simulink model "gtm_design"  (R2021b)
settings: Solver=VariableStepAuto  StartTime=0.0  StopTime=10.0  MinStep=0.00999  RelTol=1e-3
StopFcn:
  | MWSout=grabmws(bdroot);
  | MWSout.lastrun=datestr(now);
values from neighbouring files (symbols this model uses):
  knots2fps = 1.68781    [setup.m]
  s = tf('s')    [setup.m]
undefined symbols (not defined in the file or in its folder): Aero, aftfuel, aftfuel_pos, AILL, AILLC, AILR, AILRC, alpha_deg, alt0, altitude_ft, Ax_g, Ay_g, Az_g, b, beta_deg, bias, BRAKEC, Cbar, cg_pos0, cg_shift_gear, ControlMode, DamageCase, DamageModels, DamageOnsetTime, deltc, Earth, ELLIB, ELLIBC, ELLOB, ELLOBC, ELRIB, ELRIBC, ELROB, ELROBC, engl_ang, engl_pos, engr_ang, engr_pos, etas0, etas1, etasc_feedthrough, FLAPLC, FLAPLIB, FLAPLOB, FLAPRC, FLAPRIB, FLAPROB, FlightMode, FuelUsed_Init, fwdfuel, fwdfuel_pos, GEAR, GEARC, Inertia0, Inertia_shift_gear, Ixx_model, Iyy_model, Izz_model, KTAS, LandingGear ... (+66)
libraries: simulink_extras x98, LPVBlockLibrary x54, simulink_need_slupdate x30, aerolibconvert2 x27, simulink x7, aerolibtransform2 x6, uavalgslib x4, UserContent_lib x2, robotcorelib x1, uavutilslib x1
(part 8 of 9)

== system gtm_design/GTM_T2/Aero/Control Surfaces/Spoilers/InboardSpoilers ==
  alpha : Inport
  beta : Inport  Port=2
  SPLLIB : Inport  Port=3
  SPLRIB : Inport  Port=4
  Constant1 : Constant  Value=[0:5]  OutDataTypeStr=uint32
  Constant3 : Constant  Value=[0:5]  OutDataTypeStr=uint32
  Gain2 : Gain  Gain=-1
  Interpolation Using Prelookup : Interpolation_n-D  NumberOfTableDimensions=4  Table=Aero.dC6_spo.data  NumSelectionDims=1
      settings: InputPortMap=u0,u1,u2,u3,u4,u5,u6
  Interpolation Using Prelookup1 : Interpolation_n-D  NumberOfTableDimensions=4  Table=Aero.dC6_spo.data  NumSelectionDims=1
      settings: InputPortMap=u0,u1,u2,u3,u4,u5,u6
  Negate Lateral : Gain  Gain=[1 -1 1 -1 1 -1]
  Prelookup1 : PreLookup  BreakpointsData=Aero.dC6_spo.alpha  IndexSearchMethod=Linear search  BeginIndexSearchUsingPreviousIndexResult=on  ExtrapMethod=Linear
  Prelookup2 : PreLookup  BreakpointsData=Aero.dC6_spo.beta  IndexSearchMethod=Linear search  BeginIndexSearchUsingPreviousIndexResult=on  ExtrapMethod=Linear
  Prelookup3 : PreLookup  BreakpointsData=Aero.dC6_spo.spo  IndexSearchMethod=Linear search  BeginIndexSearchUsingPreviousIndexResult=on  ExtrapMethod=Linear
  Prelookup4 : PreLookup  BreakpointsData=Aero.dC6_spo.beta  IndexSearchMethod=Linear search  BeginIndexSearchUsingPreviousIndexResult=on  ExtrapMethod=Linear
  Prelookup5 : PreLookup  BreakpointsData=Aero.dC6_spo.spo  IndexSearchMethod=Linear search  BeginIndexSearchUsingPreviousIndexResult=on  ExtrapMethod=Linear
  Left : Outport
  Right : Outport  Port=2
  wires:
  Gain2/1 -> Prelookup2/1
  Negate Lateral/1 -> Left/1
  Interpolation Using Prelookup1/1 -> Right/1
  SPLRIB/1 -> Prelookup5/1
  beta/1 -> Gain2/1, Prelookup4/1
  alpha/1 -> Prelookup1/1
  SPLLIB/1 -> Prelookup3/1
  Prelookup1/1 -> Interpolation Using Prelookup/1, Interpolation Using Prelookup1/1
  Prelookup1/2 -> Interpolation Using Prelookup/2, Interpolation Using Prelookup1/2
  Prelookup2/1 -> Interpolation Using Prelookup/3
  Prelookup2/2 -> Interpolation Using Prelookup/4
  Prelookup3/1 -> Interpolation Using Prelookup/5
  Prelookup3/2 -> Interpolation Using Prelookup/6
  Constant3/1 -> Interpolation Using Prelookup/7
  Prelookup4/1 -> Interpolation Using Prelookup1/3
  Prelookup4/2 -> Interpolation Using Prelookup1/4
  Prelookup5/1 -> Interpolation Using Prelookup1/5
  Prelookup5/2 -> Interpolation Using Prelookup1/6
  Constant1/1 -> Interpolation Using Prelookup1/7
  Interpolation Using Prelookup/1 -> Negate Lateral/1

== system gtm_design/GTM_T2/Aero/Control Surfaces/Spoilers/OutboardSpoilers ==
  alpha : Inport
  beta : Inport  Port=2
  SPLLIB : Inport  Port=3
  SPLRIB : Inport  Port=4
  Constant1 : Constant  Value=[0:5]  OutDataTypeStr=uint32
  Constant3 : Constant  Value=[0:5]  OutDataTypeStr=uint32
  Gain2 : Gain  Gain=-1
  Interpolation Using Prelookup : Interpolation_n-D  NumberOfTableDimensions=4  Table=Aero.dC6_spo.data  NumSelectionDims=1
      settings: InputPortMap=u0,u1,u2,u3,u4,u5,u6
  Interpolation Using Prelookup1 : Interpolation_n-D  NumberOfTableDimensions=4  Table=Aero.dC6_spo.data  NumSelectionDims=1
      settings: InputPortMap=u0,u1,u2,u3,u4,u5,u6
  Negate Lateral : Gain  Gain=[1 -1 1 -1 1 -1]
  Prelookup1 : PreLookup  BreakpointsData=Aero.dC6_spo.alpha  IndexSearchMethod=Linear search  BeginIndexSearchUsingPreviousIndexResult=on  ExtrapMethod=Linear
  Prelookup2 : PreLookup  BreakpointsData=Aero.dC6_spo.beta  IndexSearchMethod=Linear search  BeginIndexSearchUsingPreviousIndexResult=on  ExtrapMethod=Linear
  Prelookup3 : PreLookup  BreakpointsData=Aero.dC6_spo.spo  IndexSearchMethod=Linear search  BeginIndexSearchUsingPreviousIndexResult=on  ExtrapMethod=Linear
  Prelookup4 : PreLookup  BreakpointsData=Aero.dC6_spo.beta  IndexSearchMethod=Linear search  BeginIndexSearchUsingPreviousIndexResult=on  ExtrapMethod=Linear
  Prelookup5 : PreLookup  BreakpointsData=Aero.dC6_spo.spo  IndexSearchMethod=Linear search  BeginIndexSearchUsingPreviousIndexResult=on  ExtrapMethod=Linear
  Left : Outport
  Right : Outport  Port=2
  wires:
  Interpolation Using Prelookup/1 -> Negate Lateral/1
  Constant1/1 -> Interpolation Using Prelookup1/7
  Prelookup5/2 -> Interpolation Using Prelookup1/6
  Prelookup5/1 -> Interpolation Using Prelookup1/5
  Prelookup4/2 -> Interpolation Using Prelookup1/4
  Prelookup4/1 -> Interpolation Using Prelookup1/3
  Constant3/1 -> Interpolation Using Prelookup/7
  Prelookup3/2 -> Interpolation Using Prelookup/6
  Prelookup3/1 -> Interpolation Using Prelookup/5
  Prelookup2/2 -> Interpolation Using Prelookup/4
  Prelookup2/1 -> Interpolation Using Prelookup/3
  Prelookup1/2 -> Interpolation Using Prelookup1/2, Interpolation Using Prelookup/2
  Prelookup1/1 -> Interpolation Using Prelookup1/1, Interpolation Using Prelookup/1
  SPLLIB/1 -> Prelookup3/1
  alpha/1 -> Prelookup1/1
  beta/1 -> Prelookup4/1, Gain2/1
  SPLRIB/1 -> Prelookup5/1
  Interpolation Using Prelookup1/1 -> Right/1
  Negate Lateral/1 -> Left/1
  Gain2/1 -> Prelookup2/1

== system gtm_design/GTM_T2/Aero/Dynamic Derviatives/Forced Oscillation with Damage Increments/Damage Effects-Increments ==
  alpha : Inport
  pqr : Inport  Port=2
  DamageCase : Inport  Port=3
  CY derivative increment due to rates : simulink_need_slupdate/Interpolation (n-D) using PreLookup  numDimsPopupSelect=3  explicitNumDims=2  table=squeeze(Aero.dC6_damage.ddinc.data(:,:,:,2))  interpMethod=Linear  extrapMethod=Linear  rangeErrorMode=None  NumSelectionDims=2
      settings: SourceProductBaseCode=SL
  Constant : Constant  Value=uint32(1)
  Constant1 : Constant  Value=[0:2]  OutDataTypeStr=uint32
  Data Type Conversion : DataTypeConversion  OutDataTypeStr=uint32
  PreLookup Index Search : simulink_need_slupdate/PreLookup Index Search  bpData=Aero.dC6_damage.ddinc.alpha  searchMode=Binary Search  cacheBpFlag=on  outputFlag=off  IndexDataType=uint32  extrapMode=Linear Extrapolation  rangeErrorMode=None
      settings: SourceProductBaseCode=SL
  Product : Product  RndMeth=Zero
  Subtract : Sum  Inputs=+-
  Sum of Elements : Sum  Inputs=+
  Increment : Outport
  wires:
  Subtract/1 -> CY derivative increment due to rates/2
  Data Type Conversion/1 -> Subtract/1
  Constant/1 -> Subtract/2
  Constant1/1 -> CY derivative increment due to rates/3
  PreLookup Index Search/1 -> CY derivative increment due to rates/1
  DamageCase/1 -> Data Type Conversion/1
  alpha/1 -> PreLookup Index Search/1
  CY derivative increment due to rates/1 -> Product/1
  pqr/1 -> Product/2
  Product/1 -> Sum of Elements/1
  Sum of Elements/1 -> Increment/1

== system gtm_design/GTM_T2/Aero/Dynamic Derviatives/Forced Oscillation with Damage Increments/Damage Effects-Scaling ==
  alpha : Inport
  DamageCase : Inport  Port=2
  Constant : Constant  Value=uint32(1)
  Constant1 : Constant  Value=[0:5]  OutDataTypeStr=uint32
  Constant2 : Constant  Value=[0:5]  OutDataTypeStr=uint32
  Constant3 : Constant  Value=[0:5]  OutDataTypeStr=uint32
  Constant4 : Constant  Value=uint32(1)
  Constant5 : Constant  Value=uint32(1)
  DamageCase3 : InportShadow  Port=2
  DamageCase4 : InportShadow  Port=2
  PreLookup Index Search : simulink_need_slupdate/PreLookup Index Search  bpData=Aero.dC6_damage.ddscale.alpha  searchMode=Binary Search  cacheBpFlag=on  outputFlag=off  IndexDataType=uint32  extrapMode=Linear Extrapolation  rangeErrorMode=None
      settings: SourceProductBaseCode=SL
  Subtract : Sum  Inputs=+-
  Subtract1 : Sum  Inputs=+-
  Subtract2 : Sum  Inputs=+-
  p : simulink_need_slupdate/Interpolation (n-D) using PreLookup  numDimsPopupSelect=3  explicitNumDims=2  table=squeeze(Aero.dC6_damage.ddscale.data(:,:,1,:))  interpMethod=Linear  extrapMethod=None - Clip  rangeErrorMode=None  NumSelectionDims=2
      settings: SourceProductBaseCode=SL
  q : simulink_need_slupdate/Interpolation (n-D) using PreLookup  numDimsPopupSelect=3  explicitNumDims=2  table=squeeze(Aero.dC6_damage.ddscale.data(:,:,2,:))  interpMethod=Linear  extrapMethod=None - Clip  rangeErrorMode=None  NumSelectionDims=2
      settings: SourceProductBaseCode=SL
  r : simulink_need_slupdate/Interpolation (n-D) using PreLookup  numDimsPopupSelect=3  explicitNumDims=2  table=squeeze(Aero.dC6_damage.ddscale.data(:,:,3,:))  interpMethod=Linear  extrapMethod=None - Clip  rangeErrorMode=None  NumSelectionDims=2
      settings: SourceProductBaseCode=SL
  Scaling_r : Outport
  Scaling_q : Outport  Port=2
  Scaling_p : Outport  Port=3
  wires:
  DamageCase4/1 -> Subtract2/1
  Subtract2/1 -> p/2
  DamageCase3/1 -> Subtract1/1
  Subtract1/1 -> q/2
  Constant5/1 -> Subtract2/2
  Constant4/1 -> Subtract1/2
  DamageCase/1 -> Subtract/1
  Subtract/1 -> r/2
  Constant/1 -> Subtract/2
  alpha/1 -> PreLookup Index Search/1
  r/1 -> Scaling_r/1
  PreLookup Index Search/1 -> r/1, q/1, p/1
  q/1 -> Scaling_q/1
  p/1 -> Scaling_p/1
  Constant1/1 -> r/3
  Constant2/1 -> q/3
  Constant3/1 -> p/3

== system gtm_design/GTM_T2/Aero/Dynamic Derviatives/Forced Oscillation with Damage Increments/Forced Oscillation ==
  alpha : Inport
  pqr : Inport  Port=2
  Assignment to Lateral : Assignment  IndexMode=Zero-based  IndexOptions=Index vector (dialog)  Indices=[1 3 5]  OutputSizes=[1 1]
  Assignment to Lateral1 : Assignment  IndexMode=Zero-based  IndexOptions=Index vector (dialog)  Indices=[1 3 5]  OutputSizes=[1 1]
  Assignment to Longitudinal : Assignment  IndexMode=Zero-based  IndexOptions=Index vector (dialog)  Indices=[0 2 4]  OutputSizes=[1 1]
  Constant : Constant  Value=zeros(6,1)
  Constant1 : Constant  Value=[0:2]  OutDataTypeStr=uint32
  Constant2 : Constant  Value=[0:2]  OutDataTypeStr=uint32
  Constant3 : Constant  Value=[0:2]  OutDataTypeStr=uint32
  Constant4 : Constant  Value=zeros(6,1)
  Constant5 : Constant  Value=zeros(6,1)
  Demux : Demux  Outputs=3
  PreLookup Index Search : simulink_need_slupdate/PreLookup Index Search  bpData=Aero.dC3_q.alpha  searchMode=Binary Search  cacheBpFlag=on  outputFlag=off  IndexDataType=uint32  extrapMode=Linear Extrapolation  rangeErrorMode=None
      settings: SourceProductBaseCode=SL
  PreLookup Index Search1 : simulink_need_slupdate/PreLookup Index Search  bpData=Aero.dC3_r.rhat  searchMode=Binary Search  cacheBpFlag=on  outputFlag=off  IndexDataType=uint32  extrapMode=Linear Extrapolation  rangeErrorMode=None
      settings: SourceProductBaseCode=SL
  PreLookup Index Search2 : simulink_need_slupdate/PreLookup Index Search  bpData=Aero.dC3_p.phat  searchMode=Binary Search  cacheBpFlag=on  outputFlag=off  IndexDataType=uint32  extrapMode=Linear Extrapolation  rangeErrorMode=None
      settings: SourceProductBaseCode=SL
  PreLookup Index Search3 : simulink_need_slupdate/PreLookup Index Search  bpData=Aero.dC3_q.qhat  searchMode=Binary Search  cacheBpFlag=on  outputFlag=off  IndexDataType=uint32  extrapMode=Linear Extrapolation  rangeErrorMode=None
      settings: SourceProductBaseCode=SL
  PreLookup Index Search4 : simulink_need_slupdate/PreLookup Index Search  bpData=Aero.dC3_p.alpha  searchMode=Binary Search  cacheBpFlag=on  outputFlag=off  IndexDataType=uint32  extrapMode=Linear Extrapolation  rangeErrorMode=None
      settings: SourceProductBaseCode=SL
  PreLookup Index Search5 : simulink_need_slupdate/PreLookup Index Search  bpData=Aero.dC3_r.alpha  searchMode=Binary Search  cacheBpFlag=on  outputFlag=off  IndexDataType=uint32  extrapMode=Linear Extrapolation  rangeErrorMode=None
      settings: SourceProductBaseCode=SL
  pitch : simulink_need_slupdate/Interpolation (n-D) using PreLookup  numDimsPopupSelect=3  explicitNumDims=2  table=Aero.dC3_q.data  interpMethod=Linear  extrapMethod=None - Clip  rangeErrorMode=None  NumSelectionDims=1
      settings: SourceProductBaseCode=SL
  roll : simulink_need_slupdate/Interpolation (n-D) using PreLookup  numDimsPopupSelect=3  explicitNumDims=2  table=Aero.dC3_p.data  interpMethod=Linear  extrapMethod=None - Clip  rangeErrorMode=None  NumSelectionDims=1
      settings: SourceProductBaseCode=SL
  yaw : simulink_need_slupdate/Interpolation (n-D) using PreLookup  numDimsPopupSelect=3  explicitNumDims=2  table=Aero.dC3_r.data  interpMethod=Linear  extrapMethod=None - Clip  rangeErrorMode=None  NumSelectionDims=1
      settings: SourceProductBaseCode=SL
  dC6_p : Outport
  dC6_q : Outport  Port=2
  dC6_r : Outport  Port=3
  wires:
  alpha/1 -> PreLookup Index Search4/1, PreLookup Index Search5/1, PreLookup Index Search/1
  pqr/1 -> Demux/1
  Constant1/1 -> pitch/3
  Demux/2 -> PreLookup Index Search3/1
  Demux/1 -> PreLookup Index Search2/1
  Demux/3 -> PreLookup Index Search1/1
  Constant2/1 -> roll/3
  Constant3/1 -> yaw/3
  Constant/1 -> Assignment to Longitudinal/1
  pitch/1 -> Assignment to Longitudinal/2
  roll/1 -> Assignment to Lateral/2
  Constant4/1 -> Assignment to Lateral/1
  Constant5/1 -> Assignment to Lateral1/1
  yaw/1 -> Assignment to Lateral1/2
  PreLookup Index Search1/1 -> yaw/2
  PreLookup Index Search2/1 -> roll/2
  PreLookup Index Search3/1 -> pitch/2
  Assignment to Lateral/1 -> dC6_p/1
  Assignment to Lateral1/1 -> dC6_r/1
  Assignment to Longitudinal/1 -> dC6_q/1
  PreLookup Index Search/1 -> pitch/1
  PreLookup Index Search4/1 -> roll/1
  PreLookup Index Search5/1 -> yaw/1

== system gtm_design/GTM_T2/Aero/Dynamic Derviatives/Forced Oscillation with Damage Increments/Normalize ==
  pqr : Inport
  TAS : Inport  Port=2
  AC_Params : Inport  Port=3
  Bus Selector2 : BusSelector  OutputSignals=B,Cbar,B
  Gain : Gain  Gain=2*(1.689)
  Mux : Mux  Inputs=3
  Product3 : Product  Inputs=**/  RndMeth=Zero
  Saturation1 : Saturate  UpperLimit=10000  LowerLimit=1
  pqrhat : Outport
  wires:
  Mux/1 -> Product3/2
  Bus Selector2/3 -> Mux/3  "<B>"
  Bus Selector2/2 -> Mux/2  "<Cbar>"
  Bus Selector2/1 -> Mux/1  "<B>"
  Product3/1 -> pqrhat/1
  Gain/1 -> Product3/3
  pqr/1 -> Product3/1
  Saturation1/1 -> Gain/1
  AC_Params/1 -> Bus Selector2/1
  TAS/1 -> Saturation1/1

== system gtm_design/GTM_T2/Aero/Dynamic Derviatives/Rotary Blended UnDamaged Case/Forced Oscillation ==
  alpha : Inport
  pqr : Inport  Port=2
  Assignment to Lateral : Assignment  IndexMode=Zero-based  IndexOptions=Index vector (dialog)  Indices=[1 3 5]  OutputSizes=[1 1]
  Assignment to Lateral1 : Assignment  IndexMode=Zero-based  IndexOptions=Index vector (dialog)  Indices=[1 3 5]  OutputSizes=[1 1]
  Assignment to Longitudinal : Assignment  IndexMode=Zero-based  IndexOptions=Index vector (dialog)  Indices=[0 2 4]  OutputSizes=[1 1]
  Constant : Constant  Value=zeros(6,1)
  Constant1 : Constant  Value=[0:2]  OutDataTypeStr=uint32
  Constant2 : Constant  Value=[0:2]  OutDataTypeStr=uint32
  Constant3 : Constant  Value=[0:2]  OutDataTypeStr=uint32
  Constant4 : Constant  Value=zeros(6,1)
  Constant5 : Constant  Value=zeros(6,1)
  Demux : Demux  Outputs=3
  PreLookup Index Search : simulink_need_slupdate/PreLookup Index Search  bpData=Aero.dC3_q.alpha  searchMode=Binary Search  cacheBpFlag=on  outputFlag=off  IndexDataType=uint32  extrapMode=Linear Extrapolation  rangeErrorMode=None
      settings: SourceProductBaseCode=SL
  PreLookup Index Search1 : simulink_need_slupdate/PreLookup Index Search  bpData=Aero.dC3_r.rhat  searchMode=Binary Search  cacheBpFlag=on  outputFlag=off  IndexDataType=uint32  extrapMode=Linear Extrapolation  rangeErrorMode=None
      settings: SourceProductBaseCode=SL
  PreLookup Index Search2 : simulink_need_slupdate/PreLookup Index Search  bpData=Aero.dC3_p.phat  searchMode=Binary Search  cacheBpFlag=on  outputFlag=off  IndexDataType=uint32  extrapMode=Linear Extrapolation  rangeErrorMode=None
      settings: SourceProductBaseCode=SL
  PreLookup Index Search3 : simulink_need_slupdate/PreLookup Index Search  bpData=Aero.dC3_q.qhat  searchMode=Binary Search  cacheBpFlag=on  outputFlag=off  IndexDataType=uint32  extrapMode=Linear Extrapolation  rangeErrorMode=None
      settings: SourceProductBaseCode=SL
  PreLookup Index Search4 : simulink_need_slupdate/PreLookup Index Search  bpData=Aero.dC3_p.alpha  searchMode=Binary Search  cacheBpFlag=on  outputFlag=off  IndexDataType=uint32  extrapMode=Linear Extrapolation  rangeErrorMode=None
      settings: SourceProductBaseCode=SL
  PreLookup Index Search5 : simulink_need_slupdate/PreLookup Index Search  bpData=Aero.dC3_r.alpha  searchMode=Binary Search  cacheBpFlag=on  outputFlag=off  IndexDataType=uint32  extrapMode=Linear Extrapolation  rangeErrorMode=None
      settings: SourceProductBaseCode=SL
  pitch : simulink_need_slupdate/Interpolation (n-D) using PreLookup  numDimsPopupSelect=3  explicitNumDims=2  table=Aero.dC3_q.data  interpMethod=Linear  extrapMethod=Linear  rangeErrorMode=None  NumSelectionDims=1
      settings: SourceProductBaseCode=SL
  roll : simulink_need_slupdate/Interpolation (n-D) using PreLookup  numDimsPopupSelect=3  explicitNumDims=2  table=Aero.dC3_p.data  interpMethod=Linear  extrapMethod=Linear  rangeErrorMode=None  NumSelectionDims=1
      settings: SourceProductBaseCode=SL
  yaw : simulink_need_slupdate/Interpolation (n-D) using PreLookup  numDimsPopupSelect=3  explicitNumDims=2  table=Aero.dC3_r.data  interpMethod=Linear  extrapMethod=Linear  rangeErrorMode=None  NumSelectionDims=1
      settings: SourceProductBaseCode=SL
  dC6_p : Outport
  dC6_q : Outport  Port=2
  dC6_r : Outport  Port=3
  wires:
  alpha/1 -> PreLookup Index Search4/1, PreLookup Index Search5/1, PreLookup Index Search/1
  pqr/1 -> Demux/1
  Constant1/1 -> pitch/3
  Demux/2 -> PreLookup Index Search3/1
  Demux/1 -> PreLookup Index Search2/1
  Demux/3 -> PreLookup Index Search1/1
  Constant2/1 -> roll/3
  Constant3/1 -> yaw/3
  Constant/1 -> Assignment to Longitudinal/1
  pitch/1 -> Assignment to Longitudinal/2
  roll/1 -> Assignment to Lateral/2
  Constant4/1 -> Assignment to Lateral/1
  Constant5/1 -> Assignment to Lateral1/1
  yaw/1 -> Assignment to Lateral1/2
  PreLookup Index Search1/1 -> yaw/2
  PreLookup Index Search2/1 -> roll/2
  PreLookup Index Search3/1 -> pitch/2
  Assignment to Lateral/1 -> dC6_p/1
  Assignment to Lateral1/1 -> dC6_r/1
  Assignment to Longitudinal/1 -> dC6_q/1
  PreLookup Index Search/1 -> pitch/1
  PreLookup Index Search4/1 -> roll/1
  PreLookup Index Search5/1 -> yaw/1

== system gtm_design/GTM_T2/Aero/Dynamic Derviatives/Rotary Blended UnDamaged Case/Rotary Balance ==
  alpha : Inport
  beta : Inport  Port=2
  w : Inport  Port=3
  Constant1 : Constant  Value=[0:5]  OutDataTypeStr=uint32
  PreLookup Index Search : simulink_need_slupdate/PreLookup Index Search  bpData=Aero.dC6_w.alpha  searchMode=Binary Search  cacheBpFlag=on  outputFlag=off  IndexDataType=uint32  extrapMode=Linear Extrapolation  rangeErrorMode=None
      settings: SourceProductBaseCode=SL
  PreLookup Index Search1 : simulink_need_slupdate/PreLookup Index Search  bpData=Aero.dC6_w.beta  searchMode=Binary Search  cacheBpFlag=on  outputFlag=off  IndexDataType=uint32  extrapMode=Linear Extrapolation  rangeErrorMode=None
      settings: SourceProductBaseCode=SL
  PreLookup Index Search2 : simulink_need_slupdate/PreLookup Index Search  bpData=Aero.dC6_w.what  searchMode=Binary Search  cacheBpFlag=on  outputFlag=off  IndexDataType=uint32  extrapMode=Linear Extrapolation  rangeErrorMode=None
      settings: SourceProductBaseCode=SL
  TableLookup : simulink_need_slupdate/Interpolation (n-D) using PreLookup  numDimsPopupSelect=4  explicitNumDims=2  table=Aero.dC6_w.data  interpMethod=Linear  extrapMethod=Linear  rangeErrorMode=None  NumSelectionDims=1
      settings: SourceProductBaseCode=SL
  dC6 : Outport
  wires:
  PreLookup Index Search/1 -> TableLookup/1
  beta/1 -> PreLookup Index Search1/1
  alpha/1 -> PreLookup Index Search/1
  TableLookup/1 -> dC6/1
  Constant1/1 -> TableLookup/4
  w/1 -> PreLookup Index Search2/1
  PreLookup Index Search1/1 -> TableLookup/3
  PreLookup Index Search2/1 -> TableLookup/2

== system gtm_design/GTM_T2/Sensors/Air Data/First Order Filter/Enabled Subsystem ==
  In : Inport
  tau : Inport  Port=2
  Enable : EnablePort
  Divide : Product  Inputs=*/
  Integrator : Integrator  InitialConditionSource=external  UpperSaturationLimit=POS_hi  LowerSaturationLimit=POS_lo
  Sum : Sum  Inputs=-+|  InputSameDT=on  SaturateOnIntegerOverflow=on  OutDataTypeStr=Inherit: Same as first input
  Out : Outport
  wires:
  Sum/1 -> Divide/1  "Error"
  In/1 -> Sum/2, Integrator/2
  Integrator/1 -> Out/1, Sum/1  "Y"
  tau/1 -> Divide/2
  Divide/1 -> Integrator/1  "Ydot"

== system gtm_design/GTM_T2/TransportDelay/Transport Delay on Bus/BusDelay/TimeDelay with IC feedthrough 15e-3 ==
  I : Inport
  Clock : Clock
  Switch : Switch  Criteria=u2 > Threshold  Threshold=TimeDelay
  Transport Delay : TransportDelay  DelayTime=TimeDelay
      settings: AttributesFormatString=%<DelayTime>
  O : Outport
  wires:
  I/1 -> Transport Delay/1, Switch/3
  Clock/1 -> Switch/2
  Switch/1 -> O/1
  Transport Delay/1 -> Switch/1

== system gtm_design/GTM_T2/TransportDelay/Transport Delay on Bus/BusDelay1/TimeDelay with IC feedthrough ==
  I : Inport
  Clock : Clock
  Switch : Switch  Criteria=u2 > Threshold  Threshold=TimeDelay
  Transport Delay : TransportDelay  DelayTime=TimeDelay
      settings: AttributesFormatString=%<DelayTime>
  O : Outport
  wires:
  I/1 -> Transport Delay/1, Switch/3
  Clock/1 -> Switch/2
  Switch/1 -> O/1
  Transport Delay/1 -> Switch/1

== system gtm_design/GTM_T2/TransportDelay/Transport Delay on Bus/BusDelay2/TimeDelay with IC feedthrough ==
  I : Inport
  Clock : Clock
  Switch : Switch  Criteria=u2 > Threshold  Threshold=TimeDelay
  Transport Delay : TransportDelay  DelayTime=TimeDelay
      settings: AttributesFormatString=%<DelayTime>
  O : Outport
  wires:
  I/1 -> Transport Delay/1, Switch/3
  Clock/1 -> Switch/2
  Switch/1 -> O/1
  Transport Delay/1 -> Switch/1

== system gtm_design/GTM_T2/TransportDelay/Transport Delay on Bus/BusDelay3/TimeDelay with IC feedthrough ==
  I : Inport
  Clock : Clock
  Switch : Switch  Criteria=u2 > Threshold  Threshold=TimeDelay
  Transport Delay : TransportDelay  DelayTime=TimeDelay
      settings: AttributesFormatString=%<DelayTime>
  O : Outport
  wires:
  I/1 -> Transport Delay/1, Switch/3
  Clock/1 -> Switch/2
  Switch/1 -> O/1
  Transport Delay/1 -> Switch/1

== system gtm_design/GTM_T2/TransportDelay/Transport Delay on Bus/BusDelay4/TimeDelay with IC feedthrough ==
  I : Inport
  Clock : Clock
  Switch : Switch  Criteria=u2 > Threshold  Threshold=TimeDelay
  Transport Delay : TransportDelay  DelayTime=TimeDelay
      settings: AttributesFormatString=%<DelayTime>
  O : Outport
  wires:
  I/1 -> Transport Delay/1, Switch/3
  Clock/1 -> Switch/2
  Switch/1 -> O/1
  Transport Delay/1 -> Switch/1

== system gtm_design/Guidance/Autopilot Trajectory Tracking/Orbit Following/Pose/Map 0_1 ==
  I : Inport
  Constant : Constant  Value=2*pi
  Constant1 : Constant  Value=0
  Gain : Gain  Gain=180/pi
  Sum : Sum  Inputs=|++
  ifnegadd2pi : Switch
  O : Outport
  wires:
  Gain/1 -> O/1
  Constant1/1 -> ifnegadd2pi/1
  Constant/1 -> ifnegadd2pi/3
  ifnegadd2pi/1 -> Sum/2
  Sum/1 -> Gain/1
  I/1 -> ifnegadd2pi/2, Sum/1

== system gtm_design/Guidance/Autopilot Trajectory Tracking/Orbit Following/Pose/VecNorm ==
  I : Inport
  Math Function2 : Math  Operator=sqrt  SignedPower=on  SaturateOnIntegerOverflow=on
  Product : Product  RndMeth=Zero
  Sum of Elements : Sum  Inputs=+
  O : Outport
  wires:
  Math Function2/1 -> O/1
  I/1 -> Product/1, Product/2
  Product/1 -> Sum of Elements/1
  Sum of Elements/1 -> Math Function2/1

== system gtm_design/Guidance/Autopilot Trajectory Tracking/Waypoint Following/Pose/Map 0_1 ==
  I : Inport
  Constant : Constant  Value=2*pi
  Constant1 : Constant  Value=0
  Gain : Gain  Gain=180/pi
  Sum : Sum  Inputs=|++
  ifnegadd2pi : Switch
  O : Outport
  wires:
  I/1 -> Sum/1, ifnegadd2pi/2
  Sum/1 -> Gain/1
  ifnegadd2pi/1 -> Sum/2
  Constant/1 -> ifnegadd2pi/3
  Constant1/1 -> ifnegadd2pi/1
  Gain/1 -> O/1

== system gtm_design/Guidance/Autopilot Trajectory Tracking/Waypoint Following/Pose/VecNorm ==
  I : Inport
  Math Function2 : Math  Operator=sqrt  SignedPower=on  SaturateOnIntegerOverflow=on
  Product : Product  RndMeth=Zero
  Sum of Elements : Sum  Inputs=+
  O : Outport
  wires:
  Sum of Elements/1 -> Math Function2/1
  Product/1 -> Sum of Elements/1
  I/1 -> Product/2, Product/1
  Math Function2/1 -> O/1

== system gtm_design/Control/Controller/Control Algorithm/Hinf Autopilot/Lateral-Directional Controller/Full State ==
  feedback : Inport
  Bus Selector : BusSelector  OutputSignals=AirData.beta_deg,MAG3.p_deg,MAG3.r_deg,MIDG.phi_deg
  Degrees to Radians{,1..2,6} (4 alike) : simulink_extras/Transformations/Degrees to Radians
  Mux : Mux
  x : Outport
  wires:
  feedback/1 -> Bus Selector/1
  Bus Selector/1 -> Degrees to Radians2/1  "<beta_deg>"
  Bus Selector/2 -> Degrees to Radians/1  "<p_deg>"
  Bus Selector/3 -> Degrees to Radians1/1  "<r_deg>"
  Bus Selector/4 -> Degrees to Radians6/1  "<phi_deg>"
  Degrees to Radians1/1 -> Mux/3  "r_rad"
  Degrees to Radians/1 -> Mux/2  "p_rad"
  Degrees to Radians6/1 -> Mux/4  "phi_rad"
  Degrees to Radians2/1 -> Mux/1  "bet_rad"
  Mux/1 -> x/1

== system gtm_design/Control/Controller/Control Algorithm/Hinf Autopilot/Lateral-Directional Controller/Scheduling Parameter ==
  feedback : Inport
  Add : Sum
  Bus Selector1 : BusSelector  OutputSignals=AirData.KTAS,MIDG.NAV_altitude_m,SurfacePos.FLAPLOB,SurfacePos.FLAPROB  OutputAsBus=on
  Bus to Vector : BusToVector
  Demux : Demux
  Gain : Gain  Gain=0.5
  Length Conversion : aerolibconvert2/Length Conversion  IU=m  OU=ft
  MATLAB Function : MATLAB Function  TreatAsAtomicUnit=on
  Mux : Mux  Inputs=3
  rho : Outport
  wires:
  feedback/1 -> Bus Selector1/1
  Bus Selector1/1 -> Bus to Vector/1
  Demux/3 -> Add/1
  Demux/1 -> MATLAB Function/1(tas)
  Demux/4 -> Add/2
  MATLAB Function/1(sas) -> Mux/1  "sas"
  Add/1 -> Gain/1
  Gain/1 -> Mux/3  "mor"
  Demux/2 -> Length Conversion/1  "alt"
  Bus to Vector/1 -> Demux/1
  Mux/1 -> rho/1
  Length Conversion/1 -> MATLAB Function/2(h), Mux/2

== system gtm_design/Control/Controller/Control Algorithm/Hinf Autopilot/Lateral-Directional Controller/Trim Command ==
  rho : Inport
  Constant : Constant  Value=0
  Constant1 : Constant  Value=0
  Mux : Mux  Inputs=2
  Terminator : Terminator
  r_eq : Outport
  wires:
  Constant1/1 -> Mux/2
  Constant/1 -> Mux/1
  rho/1 -> Terminator/1
  Mux/1 -> r_eq/1

== system gtm_design/Control/Controller/Control Algorithm/Hinf Autopilot/Lateral-Directional Controller/Trim Input ==
  rho : Inport
  Constant1 : Constant  Value=0
  Constant2 : Constant
  Constant3 : Constant
  LPVBlock : LPVBlockLibrary/LPVBlock  sys=sch_param.sch_aileron_trim  plist={'rho1_sas_param';'rho2_alt_param';'rho3_mor_param'}  x0=0
      settings: SourceProductName=LPVTools Blocks
  LPVBlock1 : LPVBlockLibrary/LPVBlock  sys=sch_param.sch_rudder_trim  plist={'rho1_sas_param';'rho2_alt_param';'rho3_mor_param'}  x0=0
      settings: SourceProductName=LPVTools Blocks
  Mux : Mux  Inputs=3
  x_eq : Outport
  wires:
  Constant3/1 -> LPVBlock1/1
  Mux/1 -> x_eq/1
  rho/1 -> LPVBlock/2, LPVBlock1/2
  Constant2/1 -> LPVBlock/1
  LPVBlock1/1 -> Mux/2  "delr_trim_deg"
  Constant1/1 -> Mux/3  "etaa_trim_deg"
  LPVBlock/1 -> Mux/1  "dela_trim_deg"

== system gtm_design/Control/Controller/Control Algorithm/Hinf Autopilot/Lateral-Directional Controller/Trim State ==
  rho : Inport
  Constant{1..4} (4 alike) : Constant
  Degrees to Radians{,1..3} (4 alike) : simulink_extras/Transformations/Degrees to Radians
  LPVBlock : LPVBlockLibrary/LPVBlock  sys=sch_param.sch_beta_trim  plist={'rho1_sas_param';'rho2_alt_param';'rho3_mor_param'}  x0=0
      settings: SourceProductName=LPVTools Blocks
  LPVBlock1 : LPVBlockLibrary/LPVBlock  sys=sch_param.sch_pdeg_trim  plist={'rho1_sas_param';'rho2_alt_param';'rho3_mor_param'}  x0=0
      settings: SourceProductName=LPVTools Blocks
  LPVBlock2 : LPVBlockLibrary/LPVBlock  sys=sch_param.sch_rdeg_trim  plist={'rho1_sas_param';'rho2_alt_param';'rho3_mor_param'}  x0=0
      settings: SourceProductName=LPVTools Blocks
  LPVBlock3 : LPVBlockLibrary/LPVBlock  sys=sch_param.sch_roll_trim  plist={'rho1_sas_param';'rho2_alt_param';'rho3_mor_param'}  x0=0
      settings: SourceProductName=LPVTools Blocks
  Mux : Mux
  x_eq : Outport
  wires:
  Degrees to Radians/1 -> Mux/1  "beta_trim_rad"
  Constant2/1 -> LPVBlock/1
  LPVBlock/1 -> Degrees to Radians/1  "beta_trim_deg"
  LPVBlock1/1 -> Degrees to Radians1/1  "p_trim_deg"
  Mux/1 -> x_eq/1
  Degrees to Radians1/1 -> Mux/2  "p_trim_rad"
  Constant3/1 -> LPVBlock1/1
  Constant1/1 -> LPVBlock2/1
  LPVBlock2/1 -> Degrees to Radians2/1  "r_trim_deg"
  Degrees to Radians2/1 -> Mux/3  "r_trim_rad"
  LPVBlock3/1 -> Degrees to Radians3/1  "roll_trim_deg"
  Constant4/1 -> LPVBlock3/1
  rho/1 -> LPVBlock3/2, LPVBlock2/2, LPVBlock1/2, LPVBlock/2
  Degrees to Radians3/1 -> Mux/4  "roll_trim_rad"

== system gtm_design/Control/Controller/Control Algorithm/Hinf Autopilot/Longitudinal Controller/Full State ==
  feedback : Inport
  Bus Selector : BusSelector  OutputSignals=AirData.KTAS,AirData.alpha_deg,MAG3.q_deg,MIDG.theta_deg,MIDG.NAV_altitude_m
  Degrees to Radians : simulink_extras/Transformations/Degrees to Radians
  Degrees to Radians1 : simulink_extras/Transformations/Degrees to Radians
  Degrees to Radians6 : simulink_extras/Transformations/Degrees to Radians
  Gain : Gain  Gain=knots2fps
  Length Conversion : aerolibconvert2/Length Conversion  IU=m  OU=ft
  Mux : Mux  Inputs=5
  x : Outport
  wires:
  Mux/1 -> x/1
  Bus Selector/5 -> Length Conversion/1  "<NAV_altitude_m>"
  Gain/1 -> Mux/1  "tas_fps"
  Degrees to Radians6/1 -> Mux/4  "q_rad"
  Degrees to Radians/1 -> Mux/2  "alp_rad"
  Degrees to Radians1/1 -> Mux/3  "q_rad"
  Bus Selector/4 -> Degrees to Radians6/1  "<theta_deg>"
  Bus Selector/3 -> Degrees to Radians1/1  "<q_deg>"
  Bus Selector/2 -> Degrees to Radians/1  "<alpha_deg>"
  Bus Selector/1 -> Gain/1  "<KTAS>"
  feedback/1 -> Bus Selector/1
  Length Conversion/1 -> Mux/5

== system gtm_design/Control/Controller/Control Algorithm/Hinf Autopilot/Longitudinal Controller/Scheduling Parameter ==
  feedback : Inport
  Add : Sum
  Bus Selector1 : BusSelector  OutputSignals=AirData.KTAS,MIDG.NAV_altitude_m,SurfacePos.FLAPLOB,SurfacePos.FLAPROB  OutputAsBus=on
  Bus to Vector : BusToVector
  Demux : Demux
  Gain : Gain  Gain=0.5
  Length Conversion : aerolibconvert2/Length Conversion  IU=m  OU=ft
  MATLAB Function : MATLAB Function  TreatAsAtomicUnit=on
  Mux : Mux  Inputs=3
  rho : Outport
  wires:
  Length Conversion/1 -> Mux/2, MATLAB Function/2(h)
  Mux/1 -> rho/1
  Bus to Vector/1 -> Demux/1
  Demux/2 -> Length Conversion/1  "alt"
  Gain/1 -> Mux/3  "mor"
  Add/1 -> Gain/1
  MATLAB Function/1(sas) -> Mux/1  "sas"
  Demux/4 -> Add/2
  Demux/1 -> MATLAB Function/1(tas)
  Demux/3 -> Add/1
  Bus Selector1/1 -> Bus to Vector/1
  feedback/1 -> Bus Selector1/1

== system gtm_design/Control/Controller/Control Algorithm/Hinf Autopilot/Longitudinal Controller/Trim Command ==
  rho : Inport
  Constant4 : Constant
  Constant5 : Constant
  LPVBlock1 : LPVBlockLibrary/LPVBlock  sys=sch_param.sch_alt_trim  plist={'rho1_sas_param';'rho2_alt_param';'rho3_mor_param'}  x0=0
      settings: SourceProductName=LPVTools Blocks
  LPVBlock2 : LPVBlockLibrary/LPVBlock  sys=sch_param.sch_tas_trim  plist={'rho1_sas_param';'rho2_alt_param';'rho3_mor_param'}  x0=0
      settings: SourceProductName=LPVTools Blocks
  Mux : Mux  Inputs=2
  knotstofps : Gain  Gain=knots2fps
  r_eq : Outport
  wires:
  knotstofps/1 -> Mux/1  "tas_trim_fps"
  rho/1 -> LPVBlock1/2, LPVBlock2/2
  Constant4/1 -> LPVBlock1/1
  LPVBlock1/1 -> Mux/2  "alt_trim_ft"
  LPVBlock2/1 -> knotstofps/1  "tas_trim_knot"
  Constant5/1 -> LPVBlock2/1
  Mux/1 -> r_eq/1

== system gtm_design/Control/Controller/Control Algorithm/Hinf Autopilot/Longitudinal Controller/Trim Input ==
  rho : Inport
  Constant1 : Constant
  Constant3 : Constant
  Mux : Mux  Inputs=2
  dele_trim : LPVBlockLibrary/LPVBlock  sys=sch_param.sch_elevator_trim  plist={'rho1_sas_param';'rho2_alt_param';'rho3_mor_param'}  x0=0
      settings: SourceProductName=LPVTools Blocks
  delt_trim : LPVBlockLibrary/LPVBlock  sys=sch_param.sch_throttle_trim  plist={'rho1_sas_param';'rho2_alt_param';'rho3_mor_param'}  x0=0
      settings: SourceProductName=LPVTools Blocks
  u_eq : Outport
  wires:
  Mux/1 -> u_eq/1
  Constant1/1 -> delt_trim/1
  delt_trim/1 -> Mux/1  "delt_trim_percent"
  rho/1 -> delt_trim/2, dele_trim/2
  dele_trim/1 -> Mux/2  "dele_trim_deg"
  Constant3/1 -> dele_trim/1

== system gtm_design/Control/Controller/Control Algorithm/Hinf Autopilot/Longitudinal Controller/Trim State ==
  rho : Inport
  Constant{2..6} (5 alike) : Constant
  Degrees to Radians : simulink_extras/Transformations/Degrees to Radians
  Degrees to Radians1 : simulink_extras/Transformations/Degrees to Radians
  Degrees to Radians2 : simulink_extras/Transformations/Degrees to Radians
  LPVBlock : LPVBlockLibrary/LPVBlock  sys=sch_param.sch_alp_trim  plist={'rho1_sas_param';'rho2_alt_param';'rho3_mor_param'}  x0=0
      settings: SourceProductName=LPVTools Blocks
  LPVBlock1 : LPVBlockLibrary/LPVBlock  sys=sch_param.sch_alt_trim  plist={'rho1_sas_param';'rho2_alt_param';'rho3_mor_param'}  x0=0
      settings: SourceProductName=LPVTools Blocks
  LPVBlock2 : LPVBlockLibrary/LPVBlock  sys=sch_param.sch_tas_trim  plist={'rho1_sas_param';'rho2_alt_param';'rho3_mor_param'}  x0=0
      settings: SourceProductName=LPVTools Blocks
  LPVBlock3 : LPVBlockLibrary/LPVBlock  sys=sch_param.sch_qdeg_trim  plist={'rho1_sas_param';'rho2_alt_param';'rho3_mor_param'}  x0=0
      settings: SourceProductName=LPVTools Blocks
  Mux : Mux  Inputs=5
  knotstofps : Gain  Gain=knots2fps
  sch_pitch_trim : LPVBlockLibrary/LPVBlock  sys=sch_param.sch_pitch_trim  plist={'rho1_sas_param';'rho2_alt_param';'rho3_mor_param'}  x0=0
      settings: SourceProductName=LPVTools Blocks
  x_eq : Outport
  wires:
  Constant5/1 -> LPVBlock2/1
  LPVBlock1/1 -> Mux/5  "alt_trim_deg"
  Constant4/1 -> LPVBlock1/1
  Mux/1 -> x_eq/1
  Degrees to Radians1/1 -> Mux/4  "theta_trim_rad"
  Constant3/1 -> sch_pitch_trim/1
  sch_pitch_trim/1 -> Degrees to Radians1/1  "theta_trim_deg"
  LPVBlock/1 -> Degrees to Radians/1  "alp_trim_deg"
  Constant2/1 -> LPVBlock/1
  LPVBlock2/1 -> knotstofps/1  "tas_trim_knot"
  Degrees to Radians/1 -> Mux/2  "alp_trim_rad"
  knotstofps/1 -> Mux/1  "tas_trim_fps"
  Constant6/1 -> LPVBlock3/1
  rho/1 -> LPVBlock/2, LPVBlock3/2, sch_pitch_trim/2, LPVBlock1/2, LPVBlock2/2
  LPVBlock3/1 -> Degrees to Radians2/1  "q_trim_deg"
  Degrees to Radians2/1 -> Mux/3  "q_trim_rad"

== system gtm_design/Control/Controller/Control Algorithm/Hinf CAS/Lateral-Directional Controller/Full State ==
  feedback : Inport
  Bus Selector : BusSelector  OutputSignals=AirData.beta_deg,MAG3.p_deg,MAG3.r_deg
  Degrees to Radians : simulink_extras/Transformations/Degrees to Radians
  Degrees to Radians1 : simulink_extras/Transformations/Degrees to Radians
  Degrees to Radians2 : simulink_extras/Transformations/Degrees to Radians
  Mux : Mux  Inputs=3
  x : Outport
  wires:
  Mux/1 -> x/1
  Degrees to Radians2/1 -> Mux/1  "bet_rad"
  Degrees to Radians/1 -> Mux/2  "p_rad"
  Degrees to Radians1/1 -> Mux/3  "r_rad"
  Bus Selector/3 -> Degrees to Radians1/1  "<r_deg>"
  Bus Selector/2 -> Degrees to Radians/1  "<p_deg>"
  Bus Selector/1 -> Degrees to Radians2/1  "<beta_deg>"
  feedback/1 -> Bus Selector/1

== system gtm_design/Control/Controller/Control Algorithm/Hinf CAS/Lateral-Directional Controller/Scheduling Parameter ==
  feedback : Inport
  Add : Sum
  Bus Selector1 : BusSelector  OutputSignals=AirData.KTAS,MIDG.NAV_altitude_m,SurfacePos.FLAPLOB,SurfacePos.FLAPROB  OutputAsBus=on
  Bus to Vector : BusToVector
  Demux : Demux
  Gain : Gain  Gain=0.5
  Length Conversion : aerolibconvert2/Length Conversion  IU=m  OU=ft
  MATLAB Function : MATLAB Function  TreatAsAtomicUnit=on
  Mux : Mux  Inputs=3
  rho : Outport
  wires:
  Length Conversion/1 -> Mux/2, MATLAB Function/2(h)
  Mux/1 -> rho/1
  Bus to Vector/1 -> Demux/1
  Demux/2 -> Length Conversion/1  "alt"
  Gain/1 -> Mux/3  "mor"
  Add/1 -> Gain/1
  MATLAB Function/1(sas) -> Mux/1  "sas"
  Demux/4 -> Add/2
  Demux/1 -> MATLAB Function/1(tas)
  Demux/3 -> Add/1
  Bus Selector1/1 -> Bus to Vector/1
  feedback/1 -> Bus Selector1/1

== system gtm_design/Control/Controller/Control Algorithm/Hinf CAS/Lateral-Directional Controller/Trim Command ==
  rho : Inport
  Constant : Constant  Value=0
  Constant1 : Constant  Value=0
  Degrees to Radians : simulink_extras/Transformations/Degrees to Radians
  Degrees to Radians1 : simulink_extras/Transformations/Degrees to Radians
  Mux : Mux  Inputs=2
  Terminator : Terminator
  r_eq : Outport
  wires:
  Mux/1 -> r_eq/1
  rho/1 -> Terminator/1
  Constant/1 -> Degrees to Radians/1  "bet_trim"
  Constant1/1 -> Degrees to Radians1/1  "p_trim"
  Degrees to Radians/1 -> Mux/1
  Degrees to Radians1/1 -> Mux/2

== system gtm_design/Control/Controller/Control Algorithm/Hinf CAS/Lateral-Directional Controller/Trim Input ==
  rho : Inport
  Constant1 : Constant  Value=0
  Constant2 : Constant
  Constant3 : Constant
  LPVBlock : LPVBlockLibrary/LPVBlock  sys=sch_param.sch_aileron_trim  plist={'rho1_sas_param';'rho2_alt_param';'rho3_mor_param'}  x0=0
      settings: SourceProductName=LPVTools Blocks
  LPVBlock1 : LPVBlockLibrary/LPVBlock  sys=sch_param.sch_rudder_trim  plist={'rho1_sas_param';'rho2_alt_param';'rho3_mor_param'}  x0=0
      settings: SourceProductName=LPVTools Blocks
  Mux : Mux  Inputs=3
  x_eq : Outport
  wires:
  Constant3/1 -> LPVBlock1/1
  Mux/1 -> x_eq/1
  rho/1 -> LPVBlock/2, LPVBlock1/2
  Constant2/1 -> LPVBlock/1
  LPVBlock1/1 -> Mux/2  "delr_trim_deg"
  Constant1/1 -> Mux/3  "etaa_trim_deg"
  LPVBlock/1 -> Mux/1  "dela_trim_deg"

== system gtm_design/Control/Controller/Control Algorithm/Hinf CAS/Lateral-Directional Controller/Trim State ==
  rho : Inport
  Constant1 : Constant
  Constant2 : Constant
  Constant3 : Constant
  Degrees to Radians : simulink_extras/Transformations/Degrees to Radians
  Degrees to Radians1 : simulink_extras/Transformations/Degrees to Radians
  Degrees to Radians2 : simulink_extras/Transformations/Degrees to Radians
  LPVBlock : LPVBlockLibrary/LPVBlock  sys=sch_param.sch_beta_trim  plist={'rho1_sas_param';'rho2_alt_param';'rho3_mor_param'}  x0=0
      settings: SourceProductName=LPVTools Blocks
  LPVBlock1 : LPVBlockLibrary/LPVBlock  sys=sch_param.sch_pdeg_trim  plist={'rho1_sas_param';'rho2_alt_param';'rho3_mor_param'}  x0=0
      settings: SourceProductName=LPVTools Blocks
  LPVBlock2 : LPVBlockLibrary/LPVBlock  sys=sch_param.sch_rdeg_trim  plist={'rho1_sas_param';'rho2_alt_param';'rho3_mor_param'}  x0=0
      settings: SourceProductName=LPVTools Blocks
  Mux : Mux  Inputs=3
  x_eq : Outport
  wires:
  Degrees to Radians/1 -> Mux/1  "beta_trim_rad"
  Constant2/1 -> LPVBlock/1
  LPVBlock/1 -> Degrees to Radians/1  "beta_trim_deg"
  LPVBlock1/1 -> Degrees to Radians1/1  "p_trim_deg"
  rho/1 -> LPVBlock2/2, LPVBlock1/2, LPVBlock/2
  Mux/1 -> x_eq/1
  Degrees to Radians1/1 -> Mux/2  "p_trim_rad"
  Constant3/1 -> LPVBlock1/1
  Constant1/1 -> LPVBlock2/1
  LPVBlock2/1 -> Degrees to Radians2/1  "r_trim_deg"
  Degrees to Radians2/1 -> Mux/3  "r_trim_rad"

== system gtm_design/Control/Controller/Control Algorithm/Hinf CAS/Longitudinal Controller/Full State ==
  feedback : Inport
  Bus Selector : BusSelector  OutputSignals=AirData.alpha_deg,MAG3.q_deg,MAG3.Az_g
  Degrees to Radians : simulink_extras/Transformations/Degrees to Radians
  Degrees to Radians1 : simulink_extras/Transformations/Degrees to Radians
  Mux : Mux  Inputs=3
  knotstofps : Gain  Gain=32.174
  y : Outport
  wires:
  feedback/1 -> Bus Selector/1
  Bus Selector/1 -> Degrees to Radians/1  "<alpha_deg>"
  Bus Selector/2 -> Degrees to Radians1/1  "<q_deg>"
  Bus Selector/3 -> knotstofps/1  "<Az_g>"
  Mux/1 -> y/1
  Degrees to Radians/1 -> Mux/1  "alp_rad"
  Degrees to Radians1/1 -> Mux/2  "q_rad"
  knotstofps/1 -> Mux/3  "Az_ft/s^2"

== system gtm_design/Control/Controller/Control Algorithm/Hinf CAS/Longitudinal Controller/Scheduling Parameter ==
  feedback : Inport
  Add : Sum
  Bus Selector1 : BusSelector  OutputSignals=AirData.KTAS,MIDG.NAV_altitude_m,SurfacePos.FLAPLOB,SurfacePos.FLAPROB  OutputAsBus=on
  Bus to Vector : BusToVector
  Demux : Demux
  Gain : Gain  Gain=0.5
  Length Conversion : aerolibconvert2/Length Conversion  IU=m  OU=ft
  MATLAB Function : MATLAB Function  TreatAsAtomicUnit=on
  Mux : Mux  Inputs=3
  rho : Outport
  wires:
  feedback/1 -> Bus Selector1/1
  Bus Selector1/1 -> Bus to Vector/1
  Demux/3 -> Add/1
  Demux/1 -> MATLAB Function/1(tas)
  Demux/4 -> Add/2
  MATLAB Function/1(sas) -> Mux/1  "sas"
  Add/1 -> Gain/1
  Gain/1 -> Mux/3  "mor"
  Demux/2 -> Length Conversion/1  "alt"
  Bus to Vector/1 -> Demux/1
  Mux/1 -> rho/1
  Length Conversion/1 -> MATLAB Function/2(h), Mux/2

== system gtm_design/Control/Controller/Control Algorithm/Hinf CAS/Longitudinal Controller/Trim Command ==
  rho : Inport
  Constant : Constant
  Terminator : Terminator
  knotstofps : Gain  Gain=32.174
  r_eq : Outport
  wires:
  rho/1 -> Terminator/1
  Constant/1 -> knotstofps/1
  knotstofps/1 -> r_eq/1  "r"

== system gtm_design/Control/Controller/Control Algorithm/Hinf CAS/Longitudinal Controller/Trim Input ==
  rho : Inport
  Constant3 : Constant
  dele_trim : LPVBlockLibrary/LPVBlock  sys=sch_param.sch_elevator_trim  plist={'rho1_sas_param';'rho2_alt_param';'rho3_mor_param'}  x0=0
      settings: SourceProductName=LPVTools Blocks
  u_eq : Outport
  wires:
  Constant3/1 -> dele_trim/1
  dele_trim/1 -> u_eq/1  "dele_trim_deg"
  rho/1 -> dele_trim/2

== system gtm_design/Control/Controller/Control Algorithm/Hinf CAS/Longitudinal Controller/Trim State ==
  rho : Inport
  Constant : Constant  Value=-1
  Constant2 : Constant
  Constant3 : Constant
  Degrees to Radians : simulink_extras/Transformations/Degrees to Radians
  Degrees to Radians1 : simulink_extras/Transformations/Degrees to Radians
  LPVBlock : LPVBlockLibrary/LPVBlock  sys=sch_param.sch_alp_trim  plist={'rho1_sas_param';'rho2_alt_param';'rho3_mor_param'}  x0=0
      settings: SourceProductName=LPVTools Blocks
  LPVBlock1 : LPVBlockLibrary/LPVBlock  sys=sch_param.sch_qdeg_trim  plist={'rho1_sas_param';'rho2_alt_param';'rho3_mor_param'}  x0=0
      settings: SourceProductName=LPVTools Blocks
  Mux : Mux  Inputs=3
  knotstofps : Gain  Gain=32.174
  x_eq : Outport
  wires:
  Degrees to Radians/1 -> Mux/1  "alp_trim_rad"
  Constant2/1 -> LPVBlock/1
  LPVBlock/1 -> Degrees to Radians/1  "alp_trim_deg"
  LPVBlock1/1 -> Degrees to Radians1/1  "q_trim_deg"
  rho/1 -> LPVBlock1/2, LPVBlock/2
  Mux/1 -> x_eq/1
  Constant/1 -> knotstofps/1  "az_trim_g"
  knotstofps/1 -> Mux/3  "az_trim_ft/s^2"
  Degrees to Radians1/1 -> Mux/2  "q_trim_rad"
  Constant3/1 -> LPVBlock1/1

== system gtm_design/Control/Controller/Control Algorithm/LPV Autopilot/Lateral-Directional Controller/Full State ==
  feedback : Inport
  Bus Selector : BusSelector  OutputSignals=AirData.beta_deg,MAG3.p_deg,MAG3.r_deg,MIDG.phi_deg
  Degrees to Radians{,1..2,6} (4 alike) : simulink_extras/Transformations/Degrees to Radians
  Mux : Mux
  x : Outport
  wires:
  Mux/1 -> x/1
  Degrees to Radians2/1 -> Mux/1  "bet_rad"
  Degrees to Radians6/1 -> Mux/4  "phi_rad"
  Degrees to Radians/1 -> Mux/2  "p_rad"
  Degrees to Radians1/1 -> Mux/3  "r_rad"
  Bus Selector/4 -> Degrees to Radians6/1  "<phi_deg>"
  Bus Selector/3 -> Degrees to Radians1/1  "<r_deg>"
  Bus Selector/2 -> Degrees to Radians/1  "<p_deg>"
  Bus Selector/1 -> Degrees to Radians2/1  "<beta_deg>"
  feedback/1 -> Bus Selector/1

== system gtm_design/Control/Controller/Control Algorithm/LPV Autopilot/Lateral-Directional Controller/Scheduling Parameter ==
  feedback : Inport
  Add : Sum
  Bus Selector1 : BusSelector  OutputSignals=AirData.KTAS,MIDG.NAV_altitude_m,SurfacePos.FLAPLOB,SurfacePos.FLAPROB  OutputAsBus=on
  Bus to Vector : BusToVector
  Demux : Demux
  Gain : Gain  Gain=0.5
  Length Conversion : aerolibconvert2/Length Conversion  IU=m  OU=ft
  MATLAB Function : MATLAB Function  TreatAsAtomicUnit=on
  Mux : Mux  Inputs=3
  rho : Outport
  wires:
  Length Conversion/1 -> Mux/2, MATLAB Function/2(h)
  Mux/1 -> rho/1
  Bus to Vector/1 -> Demux/1
  Demux/2 -> Length Conversion/1  "alt"
  Gain/1 -> Mux/3  "mor"
  Add/1 -> Gain/1
  MATLAB Function/1(sas) -> Mux/1  "sas"
  Demux/4 -> Add/2
  Demux/1 -> MATLAB Function/1(tas)
  Demux/3 -> Add/1
  Bus Selector1/1 -> Bus to Vector/1
  feedback/1 -> Bus Selector1/1

== system gtm_design/Control/Controller/Control Algorithm/LPV Autopilot/Lateral-Directional Controller/Trim Command ==
  rho : Inport
  Constant : Constant  Value=0
  Constant1 : Constant  Value=0
  Mux : Mux  Inputs=2
  Terminator : Terminator
  r_eq : Outport
  wires:
  Mux/1 -> r_eq/1
  rho/1 -> Terminator/1
  Constant/1 -> Mux/1
  Constant1/1 -> Mux/2

== system gtm_design/Control/Controller/Control Algorithm/LPV Autopilot/Lateral-Directional Controller/Trim Input ==
  rho : Inport
  Constant1 : Constant  Value=0
  Constant2 : Constant
  Constant3 : Constant
  LPVBlock : LPVBlockLibrary/LPVBlock  sys=sch_param.sch_aileron_trim  plist={'rho1_sas_param';'rho2_alt_param';'rho3_mor_param'}  x0=0
      settings: SourceProductName=LPVTools Blocks
  LPVBlock1 : LPVBlockLibrary/LPVBlock  sys=sch_param.sch_rudder_trim  plist={'rho1_sas_param';'rho2_alt_param';'rho3_mor_param'}  x0=0
      settings: SourceProductName=LPVTools Blocks
  Mux : Mux  Inputs=3
  x_eq : Outport
  wires:
  Constant3/1 -> LPVBlock1/1
  Mux/1 -> x_eq/1
  rho/1 -> LPVBlock/2, LPVBlock1/2
  Constant2/1 -> LPVBlock/1
  LPVBlock1/1 -> Mux/2  "delr_trim_deg"
  Constant1/1 -> Mux/3  "etaa_trim_deg"
  LPVBlock/1 -> Mux/1  "dela_trim_deg"

== system gtm_design/Control/Controller/Control Algorithm/LPV Autopilot/Lateral-Directional Controller/Trim State ==
  rho : Inport
  Constant{1..4} (4 alike) : Constant
  Degrees to Radians{,1..3} (4 alike) : simulink_extras/Transformations/Degrees to Radians
  LPVBlock : LPVBlockLibrary/LPVBlock  sys=sch_param.sch_beta_trim  plist={'rho1_sas_param';'rho2_alt_param';'rho3_mor_param'}  x0=0
      settings: SourceProductName=LPVTools Blocks
  LPVBlock1 : LPVBlockLibrary/LPVBlock  sys=sch_param.sch_pdeg_trim  plist={'rho1_sas_param';'rho2_alt_param';'rho3_mor_param'}  x0=0
      settings: SourceProductName=LPVTools Blocks
  LPVBlock2 : LPVBlockLibrary/LPVBlock  sys=sch_param.sch_rdeg_trim  plist={'rho1_sas_param';'rho2_alt_param';'rho3_mor_param'}  x0=0
      settings: SourceProductName=LPVTools Blocks
  LPVBlock3 : LPVBlockLibrary/LPVBlock  sys=sch_param.sch_roll_trim  plist={'rho1_sas_param';'rho2_alt_param';'rho3_mor_param'}  x0=0
      settings: SourceProductName=LPVTools Blocks
  Mux : Mux
  x_eq : Outport
  wires:
  Degrees to Radians/1 -> Mux/1  "beta_trim_rad"
  Constant2/1 -> LPVBlock/1
  LPVBlock/1 -> Degrees to Radians/1  "beta_trim_deg"
  LPVBlock1/1 -> Degrees to Radians1/1  "p_trim_deg"
  Mux/1 -> x_eq/1
  Degrees to Radians1/1 -> Mux/2  "p_trim_rad"
  Constant3/1 -> LPVBlock1/1
  Constant1/1 -> LPVBlock2/1
  LPVBlock2/1 -> Degrees to Radians2/1  "r_trim_deg"
  Degrees to Radians2/1 -> Mux/3  "r_trim_rad"
  LPVBlock3/1 -> Degrees to Radians3/1  "roll_trim_deg"
  Constant4/1 -> LPVBlock3/1
  rho/1 -> LPVBlock3/2, LPVBlock2/2, LPVBlock1/2, LPVBlock/2
  Degrees to Radians3/1 -> Mux/4  "roll_trim_rad"

== system gtm_design/Control/Controller/Control Algorithm/LPV Autopilot/Longitudinal Controller/Full State ==
  feedback : Inport
  Bus Selector : BusSelector  OutputSignals=AirData.KTAS,AirData.alpha_deg,MAG3.q_deg,MIDG.theta_deg,MIDG.NAV_altitude_m
  Degrees to Radians : simulink_extras/Transformations/Degrees to Radians
  Degrees to Radians1 : simulink_extras/Transformations/Degrees to Radians
  Degrees to Radians6 : simulink_extras/Transformations/Degrees to Radians
  Gain : Gain  Gain=knots2fps
  Length Conversion : aerolibconvert2/Length Conversion  IU=m  OU=ft
  Mux : Mux  Inputs=5
  x : Outport
  wires:
  Mux/1 -> x/1
  Bus Selector/5 -> Length Conversion/1  "<NAV_altitude_m>"
  Gain/1 -> Mux/1  "tas_fps"
  Degrees to Radians6/1 -> Mux/4  "q_rad"
  Degrees to Radians/1 -> Mux/2  "alp_rad"
  Degrees to Radians1/1 -> Mux/3  "q_rad"
  Bus Selector/4 -> Degrees to Radians6/1  "<theta_deg>"
  Bus Selector/3 -> Degrees to Radians1/1  "<q_deg>"
  Bus Selector/2 -> Degrees to Radians/1  "<alpha_deg>"
  Bus Selector/1 -> Gain/1  "<KTAS>"
  feedback/1 -> Bus Selector/1
  Length Conversion/1 -> Mux/5
